simulink model "nonlinearAirframe"  (R2026a)
settings: Solver=ode3  StartTime=0  FixedStep=Ts  EnableMultiTasking=on
undefined symbols (not defined in the file): initPosLLA, Vehicle
libraries: actuatorsLibrary x3, shared6dof x1
settings Model: Creator=The MathWorks, Inc.  LastModifiedBy=The MathWorks, Inc.
settings OptimizationCC: BufferReuse=off
settings HardwareCC: ProdHWDeviceType=32-bit Generic

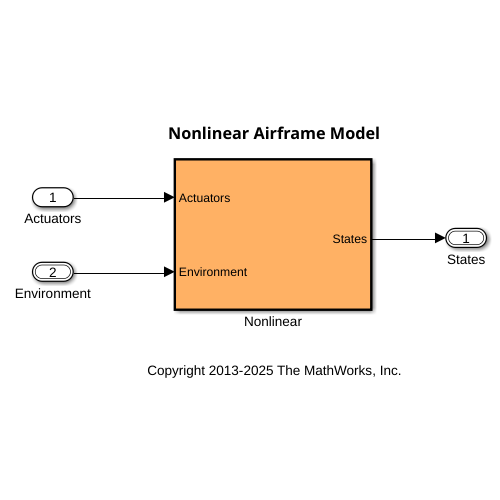
[thumbnail: Simulink's stored preview of the top-level diagram]
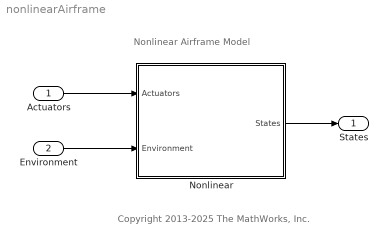
== system nonlinearAirframe ==
  note: Copyright 2013-2025 The MathWorks, Inc.
  note: Nonlinear Airframe Model
  Actuators : Inport
  Environment : Inport  Port=2  OutDataTypeStr=Bus: EnvironmentBus  BusOutputAsStruct=on
  Nonlinear : Subsystem  TreatAsAtomicUnit=on
      mask init:
      | vehicleNonlinearVars;
  States : Outport  OutDataTypeStr=Bus: StatesBus  VectorParamsAs1DForOutWhenUnconnected=off  BusOutputAsStruct=on
  wires:
  Actuators/1 -> Nonlinear/1(Actuators)
  Environment/1 -> Nonlinear/2(Environment)
  Nonlinear/1(States) -> States/1

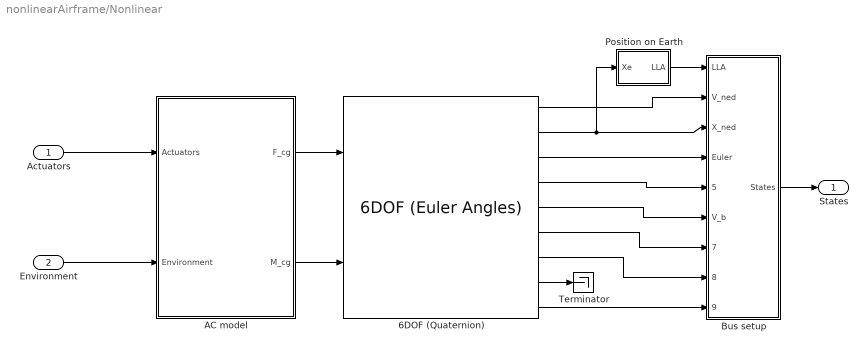
== system nonlinearAirframe/Nonlinear ==
  Actuators : Inport
  Environment : Inport  Port=2
  6DOF (Quaternion) : shared6dof/6DOF (Euler Angles)  units=Metric (MKS)  mtype=Fixed  rep=Quaternion  xme_0=initPosNED  Vm_0=initVb  eul_0=initEuler  pm_0=initAngRates  mass_0=mass  mass_e=0.5  mass_f=2.0  inertia=inertia  inertia_e=eye(3)  inertia_f=2*eye(3)  k_quat=Vehicle.Nonlinear.Nonlinear.SixDOF.quatGain  vre_flag=on  abi_flag=on  aMode=aMode  xme_statename=''  Vm_statename=''  eul_statename=''  quat_statename=''  pm_statename=''  mass_statename=''
  AC model : Subsystem
  Bus setup : Subsystem
  Position on Earth : Subsystem  Priority=1  TreatAsAtomicUnit=on
  Terminator : Terminator
  States : Outport  VectorParamsAs1DForOutWhenUnconnected=off
  wires:
  Actuators/1 -> AC model/1(Actuators)
  Environment/1 -> AC model/2(Environment)
  AC model/1(F_cg) -> 6DOF (Quaternion)/1
  AC model/2(M_cg) -> 6DOF (Quaternion)/2
  6DOF (Quaternion)/1 -> Bus setup/2(V_ned)
  6DOF (Quaternion)/2 -> Position on Earth/1(Xe), Bus setup/3(X_ned)
  6DOF (Quaternion)/3 -> Bus setup/4(Euler)
  6DOF (Quaternion)/4 -> Bus setup/5(DCM_be)
  6DOF (Quaternion)/5 -> Bus setup/6(V_b)
  6DOF (Quaternion)/6 -> Bus setup/7(Omega_b)
  6DOF (Quaternion)/7 -> Bus setup/8(dOmega_b)
  Position on Earth/1(LLA) -> Bus setup/1(LLA)
  Bus setup/1(States) -> States/1
  6DOF (Quaternion)/9 -> Bus setup/9(Accel_b)
  6DOF (Quaternion)/8 -> Terminator/1

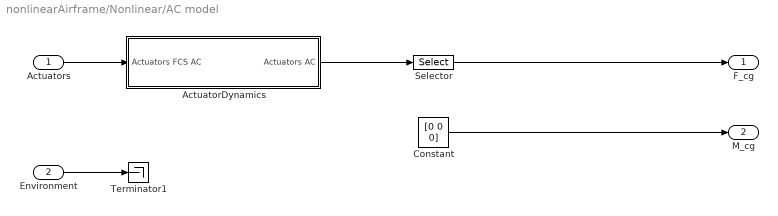
== system nonlinearAirframe/Nonlinear/AC model ==
  Actuators : Inport
  Environment : Inport  Port=2
  ActuatorDynamics : Subsystem  Variant=on
  Constant : Constant  Value=[0 0 0]
  Selector : Selector  InputPortWidth=4  IndexOptions=Index vector (dialog)  Indices=[1 2 3]  OutputSizes=1
  Terminator1 : Terminator
  F_cg : Outport  VectorParamsAs1DForOutWhenUnconnected=off
  M_cg : Outport  Port=2  VectorParamsAs1DForOutWhenUnconnected=off
  wires:
  Environment/1 -> Terminator1/1
  Selector/1 -> F_cg/1
  Actuators/1 -> ActuatorDynamics/1(Actuators FCS AC)
  ActuatorDynamics/1(Actuators AC) -> Selector/1
  Constant/1 -> M_cg/1

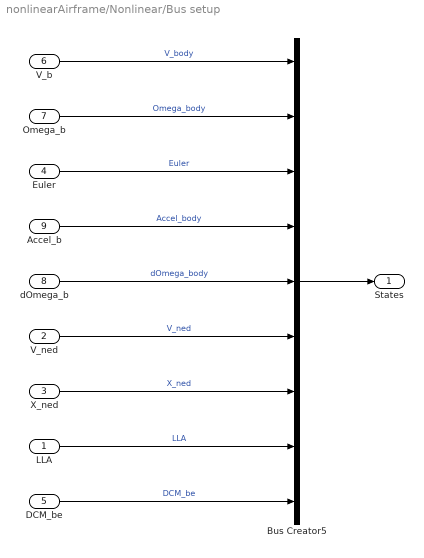
== system nonlinearAirframe/Nonlinear/Bus setup ==
  LLA : Inport  PortDimensions=3
  V_ned : Inport  Port=2  PortDimensions=3
  X_ned : Inport  Port=3  PortDimensions=3
  Euler : Inport  Port=4  PortDimensions=3
  DCM_be : Inport  Port=5  PortDimensions=[3 3]
  V_b : Inport  Port=6  PortDimensions=3
  Omega_b : Inport  Port=7  PortDimensions=3
  dOmega_b : Inport  Port=8  PortDimensions=3
  Accel_b : Inport  Port=9  PortDimensions=3
  Bus Creator5 : BusCreator  Inputs=9  OutDataTypeStr=Bus: StatesBus  NonVirtualBus=on
  States : Outport  VectorParamsAs1DForOutWhenUnconnected=off
  wires:
  Bus Creator5/1 -> States/1
  V_b/1 -> Bus Creator5/1  "V_body"
  Omega_b/1 -> Bus Creator5/2  "Omega_body"
  Euler/1 -> Bus Creator5/3  "Euler"
  X_ned/1 -> Bus Creator5/7  "X_ned"
  Accel_b/1 -> Bus Creator5/4  "Accel_body"
  LLA/1 -> Bus Creator5/8  "LLA"
  dOmega_b/1 -> Bus Creator5/5  "dOmega_body"
  DCM_be/1 -> Bus Creator5/9  "DCM_be"
  V_ned/1 -> Bus Creator5/6  "V_ned"

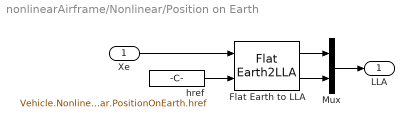
== system nonlinearAirframe/Nonlinear/Position on Earth ==
  Xe : Inport
  Flat Earth to LLA : FlatEarth2LLA  R=6378137  LL0=initPosLLA(1:2)  psi=Vehicle.Nonlinear.Nonlinear.PositionOnEarth.FlatEarthToLLA.xAxis
  Mux : Mux  Inputs=2
  href : Constant  Value=Vehicle.Nonlinear.Nonlinear.PositionOnEarth.href
  LLA : Outport  VectorParamsAs1DForOutWhenUnconnected=off
  wires:
  Mux/1 -> LLA/1
  Xe/1 -> Flat Earth to LLA/1
  Flat Earth to LLA/1 -> Mux/1
  Flat Earth to LLA/2 -> Mux/2
  href/1 -> Flat Earth to LLA/2

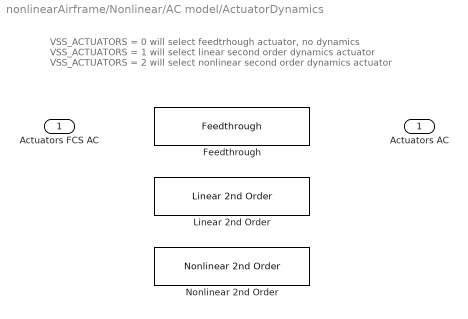
== system nonlinearAirframe/Nonlinear/AC model/ActuatorDynamics ==
  note: VSS_ACTUATORS = 0 will select feedtrhough actuator, no dynamics
      | VSS_ACTUATORS = 1 will select linear second order dynamics actuator
      | VSS_ACTUATORS = 2 will select nonlinear second order dynamics actuator
  Actuators FCS AC : Inport
  Feedthrough : actuatorsLibrary/Feedthrough  SystemSampleTime=-1  VariantControl=VSS_ACTUATORS_FEEDTHROUGH  VariantActivationTime=update diagram  EmptyChoice=off  PassThrough=off  PassThroughVariantControl=(default)  EmptyChoiceVariantControl=(default)  AllowFlexibleInterface=on  Latency=0  AutoFrameSizeCalculation=off
  Linear 2nd Order : actuatorsLibrary/Linear 2nd Order  SystemSampleTime=-1  VariantControl=VSS_ACTUATORS_LINEAR  VariantActivationTime=update diagram  EmptyChoice=off  PassThrough=off  PassThroughVariantControl=(default)  EmptyChoiceVariantControl=(default)  AllowFlexibleInterface=on  Latency=0  AutoFrameSizeCalculation=off
  Nonlinear 2nd Order : actuatorsLibrary/Nonlinear 2nd Order  SystemSampleTime=-1  VariantControl=VSS_ACTUATORS_NONLINEAR  VariantActivationTime=update diagram  EmptyChoice=off  PassThrough=off  PassThroughVariantControl=(default)  EmptyChoiceVariantControl=(default)  AllowFlexibleInterface=on  Latency=0  AutoFrameSizeCalculation=off
  Actuators AC : Outport  VectorParamsAs1DForOutWhenUnconnected=off
